simulink model "simulinkPID"  (R2019a)
settings: Solver=VariableStepAuto  StartTime=0.0  StopTime=10  RelTol=1e-3
values from neighbouring files (symbols this model uses):
  A = [5.0; 5.0; 0.5]    [SCARA_Init.m]
  B = [0.5; 0.5; 0.02]    [SCARA_Init.m]
  C = [27.5; 27.5; 0.7]    [SCARA_Init.m]
  f = [0.01; 0.01; 0.05]    [SCARA_Init.m]
  g_vec = [0, 0, -g, 0]    [SCARA_Init.m]
  J1 = [ (1/6)*m1*L1^2, 0, 0, m1*(L1/2) ... (first row only)    [SCARA_Init.m]
  J2 = [ (1/6)*m2*L2^2, 0, 0, m2*(L2/2) ... (first row only)    [SCARA_Init.m]
  L1 = 0.45    [SCARA_Init.m]
  L2 = 0.35    [SCARA_Init.m]
  L3 = 0.5    [SCARA_Init.m]
  m1 = 14    [SCARA_Init.m]
  m2 = 18    [SCARA_Init.m]
  m3 = 2    [SCARA_Init.m]
  r = 0.02    [SCARA_Init.m]
  rc1 = [L1/2; 0; 0; 1]    [SCARA_Init.m]
  rc2 = [L2/2; 0; 0; 1]    [SCARA_Init.m]
settings Model: Creator=bahaa  LastModifiedBy=bahaa

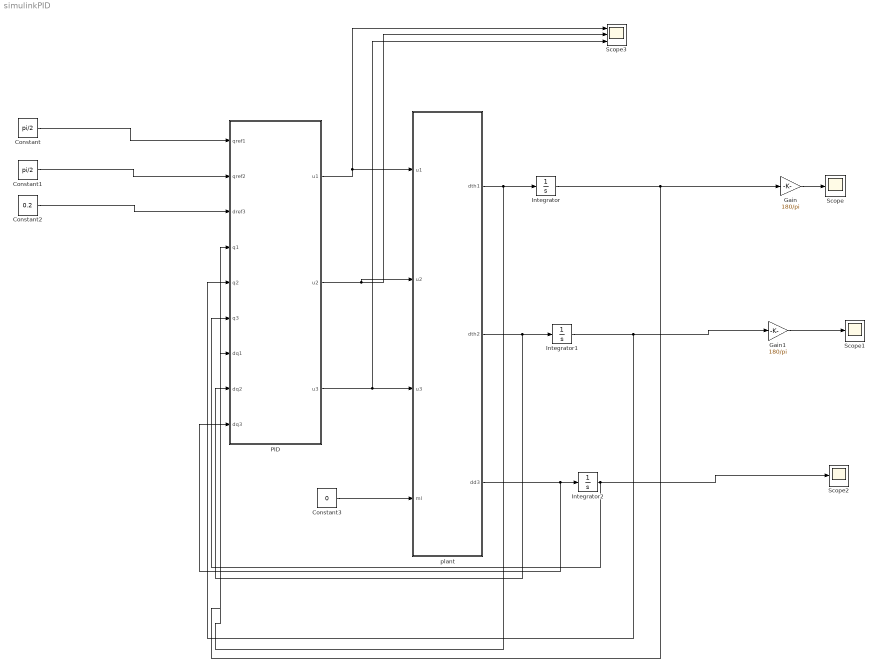
== system simulinkPID ==
  Constant : Constant  Value=pi/2
  Constant1 : Constant  Value=pi/2
  Constant2 : Constant  Value=0.2
  Constant3 : Constant  Value=0
  Gain : Gain  Gain=180/pi
  Gain1 : Gain  Gain=180/pi
  Integrator : Integrator
  Integrator1 : Integrator
  Integrator2 : Integrator
  PID : MATLAB Function  TreatAsAtomicUnit=on  SystemSampleTime=0.001
  Scope : Scope
  Scope1 : Scope
  Scope2 : Scope
  Scope3 : Scope  NumInputPorts=3
  plant : Subsystem
  wires:
  plant/1(dth1) -> PID/7(dq1), Integrator/1
  plant/2(dth2) -> PID/8(dq2), Integrator1/1
  plant/3(dd3) -> PID/9(dq3), Integrator2/1
  PID/1(u1) -> Scope3/1, plant/1(u1)
  PID/2(u2) -> Scope3/2, plant/2(u2)
  PID/3(u3) -> Scope3/3, plant/3(u3)
  Integrator/1 -> PID/4(q1), Gain/1
  Integrator1/1 -> PID/5(q2), Gain1/1
  Integrator2/1 -> PID/6(q3), Scope2/1
  Constant2/1 -> PID/3(dref3)
  Constant1/1 -> PID/2(qref2)
  Constant/1 -> PID/1(qref1)
  Constant3/1 -> plant/4(ml)
  Gain/1 -> Scope/1
  Gain1/1 -> Scope1/1

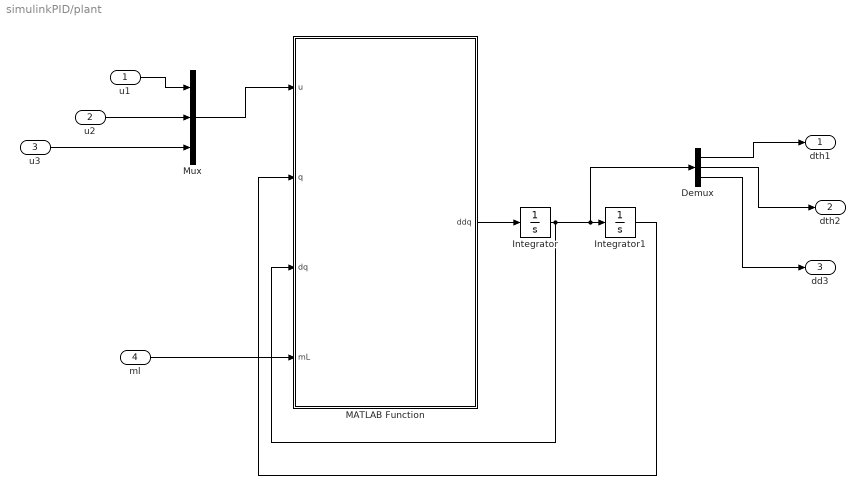
== system simulinkPID/plant ==
  u1 : Inport
  u2 : Inport  Port=2
  u3 : Inport  Port=3
  ml : Inport  Port=4
  Demux : Demux  Outputs=3
  Integrator : Integrator  InitialCondition=[0;0;0]
  Integrator1 : Integrator  InitialCondition=[0;0;0]
  MATLAB Function : MATLAB Function  TreatAsAtomicUnit=on
  Mux : Mux  Inputs=3
  dth1 : Outport
  dth2 : Outport  Port=2
  dd3 : Outport  Port=3
  wires:
  Integrator1/1 -> MATLAB Function/2(q)
  MATLAB Function/1(ddq) -> Integrator/1
  Mux/1 -> MATLAB Function/1(u)
  Integrator/1 -> MATLAB Function/3(dq), Demux/1, Integrator1/1
  u2/1 -> Mux/2
  Demux/1 -> dth1/1
  ml/1 -> MATLAB Function/4(mL)
  u1/1 -> Mux/1
  u3/1 -> Mux/3
  Demux/2 -> dth2/1
  Demux/3 -> dd3/1

== matlab function simulinkPID/PID ==
  data: qref1 input; u1 output; qref2 input; dref3 input; q1 input; q2 input; q3 input; dq1 input; dq2 input; dq3 input; u2 output; u3 output
function [u1, u2, u3] = scara_pid_controller(qref1, qref2, dref3, q1, q2, q3, dq1, dq2, dq3)

% خطوة المحاكاة الزمنية
    dt = 0.001; 
    Kp1 = 13; 
    Ki1 = 0; 
    Kd1 = 8;
    
    Kp2 = 13; 
    Ki2 = 0; 
    Kd2 =6;
   
    Kp3 =18; 
    Ki3 =0 ; 
    Kd3 = 13;
     
    
    persistent e_integral1 e_integral2 e_integral3;
    if isempty(e_integral1)
        e_integral1 = 0;
    end
    if isempty(e_integral2)
        e_integral2 = 0;
    end
    if isempty(e_integral3)
        e_integral3 = 0;
    end

% J1

    e1 = qref1 - q1;                           
    e_integral1 = e_integral1 + (e1 * dt);     
    e_derivative1 = 0 - dq1;                   
    
    u1 = (Kp1 * e1) + (Ki1 * e_integral1) + (Kd1 * e_derivative1); 

% J2
 
    e2 = qref2 - q2;                           
    e_integral2 = e_integral2 + (e2*dt);     
    e_derivative2 = 0 - dq2;                   
    
    u2 = (Kp2 * e2) + (Ki2 * e_integral2) + (Kd2 * e_derivative2); 
% J3
  
    e3 = dref3 - q3;                           
    e_integral3 = e_integral3 + (e3 * dt);     
    e_derivative3 = 0 - dq3;
    
    
    u_pid3 = (Kp3 * e3) + (Ki3 * e_integral3) + (Kd3 * e_derivative3); 
    

    m3 = 2;         
   
    g = 9.81;       
    A3 = 0.5;       % ثابت المحرك
    
    u_gravity = - (m3 * g) / A3; % الجهد الثابت لتعليق الذراع
    
  
    u3 = u_pid3 + u_gravity;
    
end

== matlab function simulinkPID/plant/MATLAB Function ==
  data: u input; ddq output; q input; dq input; mL input; g_vec parameter; f parameter; C parameter; B parameter; A parameter; J2 parameter; J1 parameter; rc2 parameter; rc1 parameter; m3 parameter; m2 parameter; m1 parameter; r parameter; L3 parameter; L2 parameter; L1 parameter
function ddq = scara_plant_numerical(u, q, dq, mL, g_vec, f, C, B, A, J2, J1, rc2, rc1, m3, m2, m1, r, L3, L2, L1)
    
    %المداخل المتغيرة u q dq mL
  
    %الزوايا
    th1 = q(1); 
    th2 = q(2);
    d3  = q(3);
    %% 1. حساب المتغيرات المعتمدة على الحمل (mL) اللحظ
%حساب كل المتغيرات التي تعتمد على تغير الحمل mL
    m3_star = m3 + mL;%كتلة الوصلة الثالثة بعد اضافة الحمل 
    zc3_star = (m3*(L3/2) + mL*L3) / m3_star;
    rc3 = [0; 0; -zc3_star; 1]; %مركز الثقل الجديد للوصلة الثالثة بعد اضافة الحمل 
    
    h3 = abs(zc3_star - (L3/2));%الازاحة بين مركز الثقل القديم والجديد للوصلة
    hL = abs(L3 - zc3_star);%الازاحة  للححمل 
    I_xx3_star = (1/12)*m3*L3^2 + m3*h3^2 + mL*hL^2;
    
    % مصفوفة J3
    J3 = [ (1/2)*m3*r^2, 0, 0, 0;
           0, (1/2)*m3*r^2, 0, 0;
           0, 0, (2*I_xx3_star - (1/2)*m3*r^2), -m3_star*zc3_star;
           0, 0, -m3_star*zc3_star, m3_star ];


    % حساب Uij
   
    A1 = [cos(th1), -sin(th1), 0, L1*cos(th1);
          sin(th1),  cos(th1), 0, L1*sin(th1);
          0,         0,        1, 0;
          0,         0,        0, 1];

    A2 = [cos(th2),  sin(th2), 0, L2*cos(th2);
          sin(th2), -cos(th2), 0, L2*sin(th2);
          0,         0,       -1, 0;
          0,         0,        0, 1];

    A3 = [1, 0, 0, 0;
          0, 1, 0, 0;
          0, 0, 1, d3;
          0, 0, 0, 1];

    
    T01 = A1;
    T02 = T01 * A2;
    T03 = T02 * A3;

    
    %الدوراني 
    Q_rev = [0, -1, 0, 0;
             1,  0, 0, 0;
             0,  0, 0, 0;
             0,  0, 0, 0];
   %الانسحابي
    Q_pris = [0, 0, 0, 0;
              0, 0, 0, 0;
              0, 0, 0, 1;
              0, 0, 0, 0];

    U11 = Q_rev * T01;
    U12 = Q_rev * T02;
    U13 = Q_rev * T03;   
    U22 = T01 * Q_rev * A2;
    U23 = T01 * Q_rev * (A2 * A3);
    U33 = T02 * Q_pris * A3;

%Dij حساب 
    D11 = trace(U11*J1*U11') + trace(U12*J2*U12') + trace(U13*J3*U13');
    D12 = trace(U12*J2*U22') + trace(U13*J3*U23'); 
    D21 = D12; % المصفوفة متناظرة
    D22 = trace(U22*J2*U22') + trace(U23*J3*U23');
    D33 = trace(U33*J3*U33');

%حساب Di 
    D_grav = zeros(3,1);
    D_grav(1) = -m1*(g_vec * U11 * rc1) - m2*(g_vec * U12 * rc2) - m3_star*(g_vec * U13 * rc3);
    D_grav(2) = -m2*(g_vec * U22 * rc2) - m3_star*(g_vec * U23 * rc3);
    D_grav(3) = -m3_star*(g_vec * U33 * rc3);

% هذه المصفوفة حصلنا عليها بعد ان عزلنا اعلى مشتق
    M = zeros(3,3);
    M(1,1) = D11 + B(1);
    M(1,2) = D12;
    M(2,1) = D21;
    M(2,2) = D22 + B(2);
    M(3,3) = D33 + B(3);

    R_vec = zeros(3,1);
    R_vec(1) = (f(1) + C(1)) * dq(1);
    R_vec(2) = (f(2) + C(2)) * dq(2);
    R_vec(3) = (f(3) + C(3)) * dq(3);

    Tau_actuator = [A(1)*u(1); A(2)*u(2); A(3)*u(3)];
    RHS = Tau_actuator - R_vec - D_grav;

    ddq = M \ RHS; % حساب أعلى مشتق
end
